simulink model "SiHADIR_Architecture"  (R2026a)
settings: Solver=VariableStepAuto
settings Model: DataDictionary=SiHADIR_Architecture_Interfaces.sldd  LastModifiedBy=Asus

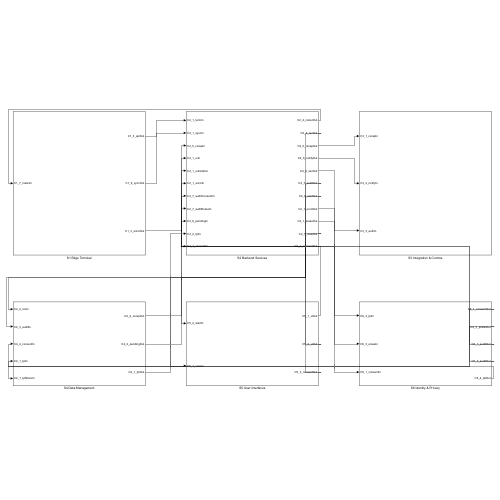
[thumbnail: Simulink's stored preview of the top-level diagram]
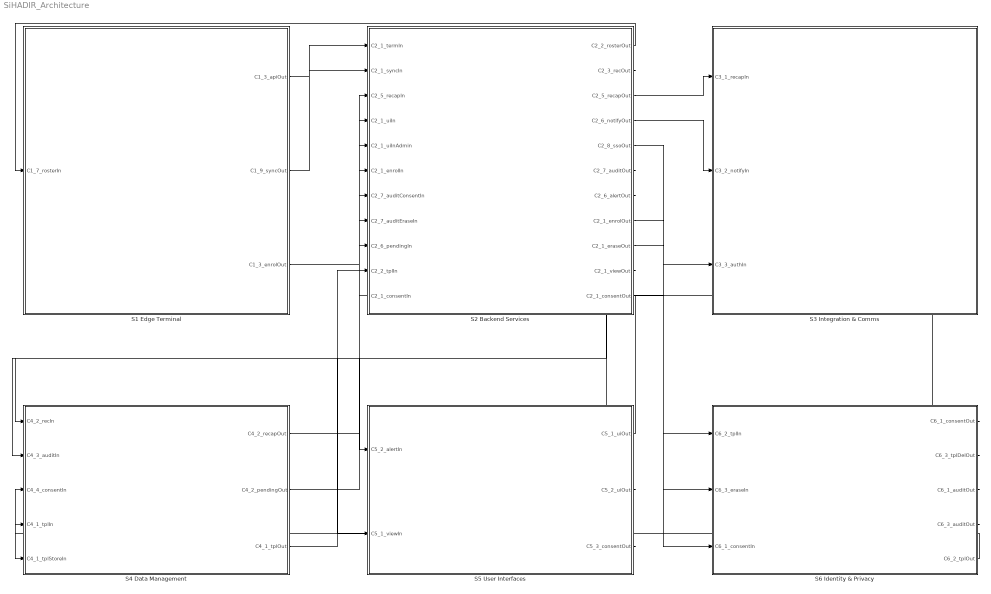
== system SiHADIR_Architecture ==
  S1 Edge Terminal : Subsystem  Description=Subsistem S1 | 11 komponen: C1.1, C1.2, C1.3, C1.4, C1.5, C1.6, C1.7, C1.8, C1.9, C1.10, C1.11
  S2 Backend Services : Subsystem  Description=Subsistem S2 | 8 komponen: C2.1, C2.2, C2.3, C2.4, C2.5, C2.6, C2.7, C2.8
  S3 Integration & Comms : Subsystem  Description=Subsistem S3 | 3 komponen: C3.1, C3.2, C3.3
  S4 Data Management : Subsystem  Description=Subsistem S4 | 4 komponen: C4.1, C4.2, C4.3, C4.4
  S5 User Interfaces : Subsystem  Description=Subsistem S5 | 3 komponen: C5.1, C5.2, C5.3
  S6 Identity & Privacy : Subsystem  Description=Subsistem S6 | 3 komponen: C6.1, C6.2, C6.3
  wires:
  S1 Edge Terminal/1(C1_3_apiOut) -> S2 Backend Services/1(C2_1_termIn)
  S1 Edge Terminal/2(C1_9_syncOut) -> S2 Backend Services/2(C2_1_syncIn)
  S2 Backend Services/1(C2_2_rosterOut) -> S1 Edge Terminal/1(C1_7_rosterIn)
  S2 Backend Services/2(C2_3_recOut) -> S4 Data Management/1(C4_2_recIn)
  S4 Data Management/1(C4_2_recapOut) -> S2 Backend Services/3(C2_5_recapIn)
  S2 Backend Services/3(C2_5_recapOut) -> S3 Integration & Comms/1(C3_1_recapIn)
  S2 Backend Services/4(C2_6_notifyOut) -> S3 Integration & Comms/2(C3_2_notifyIn)
  S2 Backend Services/5(C2_8_ssoOut) -> S3 Integration & Comms/3(C3_3_authIn)
  S2 Backend Services/6(C2_7_auditOut) -> S4 Data Management/2(C4_3_auditIn)
  S5 User Interfaces/1(C5_1_uiOut) -> S2 Backend Services/4(C2_1_uiIn)
  S5 User Interfaces/2(C5_2_uiOut) -> S2 Backend Services/5(C2_1_uiInAdmin)
  S6 Identity & Privacy/1(C6_1_consentOut) -> S4 Data Management/3(C4_4_consentIn)
  S6 Identity & Privacy/2(C6_3_tplDelOut) -> S4 Data Management/4(C4_1_tplIn)
  S1 Edge Terminal/3(C1_3_enrolOut) -> S2 Backend Services/6(C2_1_enrolIn)
  S6 Identity & Privacy/3(C6_1_auditOut) -> S2 Backend Services/7(C2_7_auditConsentIn)
  S6 Identity & Privacy/4(C6_3_auditOut) -> S2 Backend Services/8(C2_7_auditEraseIn)
  S4 Data Management/2(C4_2_pendingOut) -> S2 Backend Services/9(C2_6_pendingIn)
  S2 Backend Services/7(C2_6_alertOut) -> S5 User Interfaces/1(C5_2_alertIn)
  S2 Backend Services/8(C2_1_enrolOut) -> S6 Identity & Privacy/1(C6_2_tplIn)
  S6 Identity & Privacy/5(C6_2_tplOut) -> S4 Data Management/5(C4_1_tplStoreIn)
  S4 Data Management/3(C4_1_tplOut) -> S2 Backend Services/10(C2_2_tplIn)
  S2 Backend Services/9(C2_1_eraseOut) -> S6 Identity & Privacy/2(C6_3_eraseIn)
  S2 Backend Services/10(C2_1_viewOut) -> S5 User Interfaces/2(C5_1_viewIn)
  S5 User Interfaces/3(C5_3_consentOut) -> S2 Backend Services/11(C2_1_consentIn)
  S2 Backend Services/11(C2_1_consentOut) -> S6 Identity & Privacy/3(C6_1_consentIn)

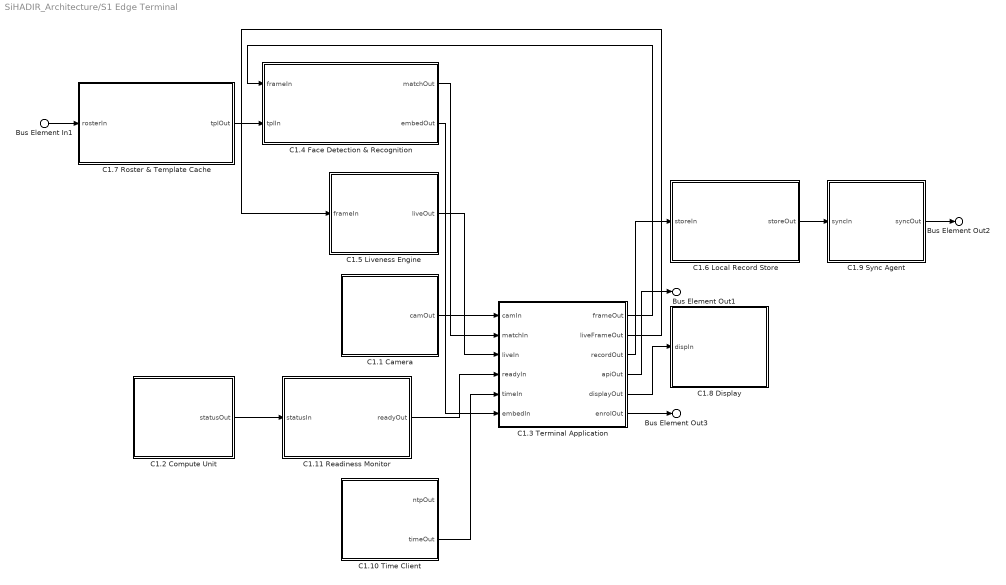
== system SiHADIR_Architecture/S1 Edge Terminal ==
  Bus Element In1 : Inport  PortName=C1_7_rosterIn
  C1.1 Camera : Subsystem  Description=ID=C1.1 | jenis=HW | fungsi=F2.1
  C1.10 Time Client : Subsystem  Description=ID=C1.10 | jenis=SW | fungsi=F12
  C1.11 Readiness Monitor : Subsystem  Description=ID=C1.11 | jenis=SW | fungsi=F11
  C1.2 Compute Unit : Subsystem  Description=ID=C1.2 | jenis=HW | fungsi=F2.2,F2.3,F2.4,F2.5,F11
  C1.3 Terminal Application : Subsystem  Description=ID=C1.3 | jenis=SW | fungsi=F3,F10
  C1.4 Face Detection & Recognition : Subsystem  Description=ID=C1.4 | jenis=SW/ML | fungsi=F2.2,F2.4,F2.5
  C1.5 Liveness Engine : Subsystem  Description=ID=C1.5 | jenis=SW/ML | fungsi=F2.3
  C1.6 Local Record Store : Subsystem  Description=ID=C1.6 | jenis=SW | fungsi=F4.2
  C1.7 Roster & Template Cache : Subsystem  Description=ID=C1.7 | jenis=SW | fungsi=F1.1,F2.5
  C1.8 Display : Subsystem  Description=ID=C1.8 | jenis=HW/SW | fungsi=F10
  C1.9 Sync Agent : Subsystem  Description=ID=C1.9 | jenis=SW | fungsi=F4.3
  Bus Element Out1 : Outport  PortName=C1_3_apiOut
  Bus Element Out2 : Outport  Port=2  PortName=C1_9_syncOut
  Bus Element Out3 : Outport  Port=3  PortName=C1_3_enrolOut
  wires:
  C1.6 Local Record Store/1(storeOut) -> C1.9 Sync Agent/1(syncIn)
  Bus Element In1/1 -> C1.7 Roster & Template Cache/1(rosterIn)
  C1.1 Camera/1(camOut) -> C1.3 Terminal Application/1(camIn)
  C1.5 Liveness Engine/1(liveOut) -> C1.3 Terminal Application/3(liveIn)
  C1.7 Roster & Template Cache/1(tplOut) -> C1.4 Face Detection & Recognition/2(tplIn)
  C1.2 Compute Unit/1(statusOut) -> C1.11 Readiness Monitor/1(statusIn)
  C1.11 Readiness Monitor/1(readyOut) -> C1.3 Terminal Application/4(readyIn)
  C1.4 Face Detection & Recognition/1(matchOut) -> C1.3 Terminal Application/2(matchIn)
  C1.4 Face Detection & Recognition/2(embedOut) -> C1.3 Terminal Application/6(embedIn)
  C1.10 Time Client/2(timeOut) -> C1.3 Terminal Application/5(timeIn)
  C1.3 Terminal Application/1(frameOut) -> C1.4 Face Detection & Recognition/1(frameIn)
  C1.3 Terminal Application/2(liveFrameOut) -> C1.5 Liveness Engine/1(frameIn)
  C1.3 Terminal Application/5(displayOut) -> C1.8 Display/1(dispIn)
  C1.3 Terminal Application/3(recordOut) -> C1.6 Local Record Store/1(storeIn)
  C1.3 Terminal Application/4(apiOut) -> Bus Element Out1/1
  C1.3 Terminal Application/6(enrolOut) -> Bus Element Out3/1
  C1.9 Sync Agent/1(syncOut) -> Bus Element Out2/1

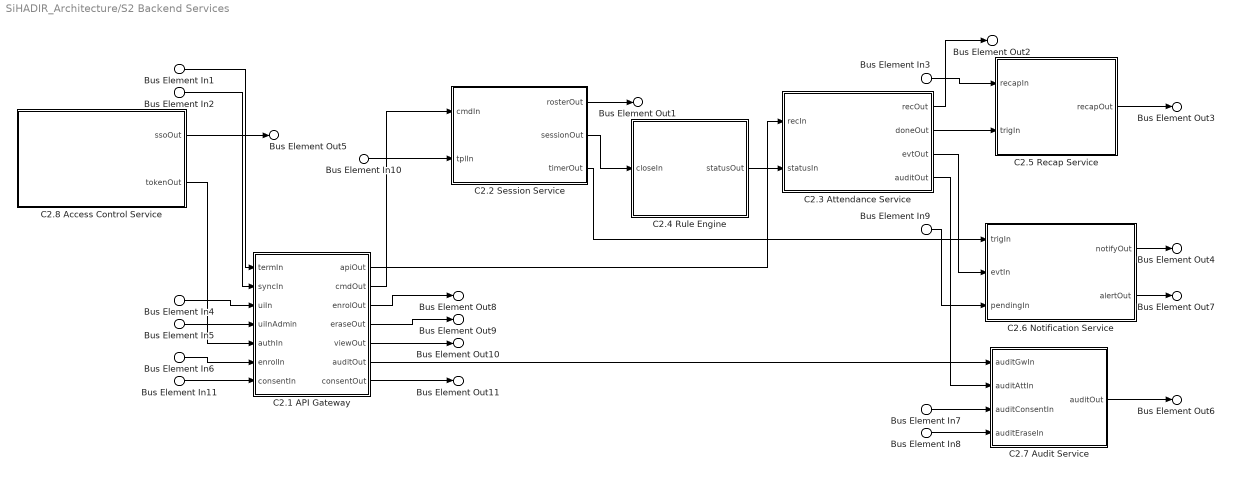
== system SiHADIR_Architecture/S2 Backend Services ==
  Bus Element In1 : Inport  PortName=C2_1_termIn
  Bus Element In2 : Inport  Port=2  PortName=C2_1_syncIn
  Bus Element In3 : Inport  Port=3  PortName=C2_5_recapIn
  Bus Element In4 : Inport  Port=4  PortName=C2_1_uiIn
  Bus Element In5 : Inport  Port=5  PortName=C2_1_uiInAdmin
  Bus Element In6 : Inport  Port=6  PortName=C2_1_enrolIn
  Bus Element In7 : Inport  Port=7  PortName=C2_7_auditConsentIn
  Bus Element In8 : Inport  Port=8  PortName=C2_7_auditEraseIn
  Bus Element In9 : Inport  Port=9  PortName=C2_6_pendingIn
  Bus Element In10 : Inport  Port=10  PortName=C2_2_tplIn
  Bus Element In11 : Inport  Port=11  PortName=C2_1_consentIn
  C2.1 API Gateway : Subsystem  Description=ID=C2.1 | jenis=SW | fungsi=F8.2
  C2.2 Session Service : Subsystem  Description=ID=C2.2 | jenis=SW | fungsi=F1.1,F1.2
  C2.3 Attendance Service : Subsystem  Description=ID=C2.3 | jenis=SW | fungsi=F4.1
  C2.4 Rule Engine : Subsystem  Description=ID=C2.4 | jenis=SW | fungsi=F3
  C2.5 Recap Service : Subsystem  Description=ID=C2.5 | jenis=SW | fungsi=F5.1,F5.2
  C2.6 Notification Service : Subsystem  Description=ID=C2.6 | jenis=SW | fungsi=F6.1,F6.2
  C2.7 Audit Service : Subsystem  Description=ID=C2.7 | jenis=SW | fungsi=F9
  C2.8 Access Control Service : Subsystem  Description=ID=C2.8 | jenis=SW | fungsi=F8.1
  Bus Element Out1 : Outport  PortName=C2_2_rosterOut
  Bus Element Out2 : Outport  Port=2  PortName=C2_3_recOut
  Bus Element Out3 : Outport  Port=3  PortName=C2_5_recapOut
  Bus Element Out4 : Outport  Port=4  PortName=C2_6_notifyOut
  Bus Element Out5 : Outport  Port=5  PortName=C2_8_ssoOut
  Bus Element Out6 : Outport  Port=6  PortName=C2_7_auditOut
  Bus Element Out7 : Outport  Port=7  PortName=C2_6_alertOut
  Bus Element Out8 : Outport  Port=8  PortName=C2_1_enrolOut
  Bus Element Out9 : Outport  Port=9  PortName=C2_1_eraseOut
  Bus Element Out10 : Outport  Port=10  PortName=C2_1_viewOut
  Bus Element Out11 : Outport  Port=11  PortName=C2_1_consentOut
  wires:
  Bus Element In2/1 -> C2.1 API Gateway/2(syncIn)
  Bus Element In4/1 -> C2.1 API Gateway/3(uiIn)
  Bus Element In6/1 -> C2.1 API Gateway/6(enrolIn)
  Bus Element In3/1 -> C2.5 Recap Service/1(recapIn)
  Bus Element In1/1 -> C2.1 API Gateway/1(termIn)
  Bus Element In5/1 -> C2.1 API Gateway/4(uiInAdmin)
  Bus Element In7/1 -> C2.7 Audit Service/3(auditConsentIn)
  Bus Element In9/1 -> C2.6 Notification Service/3(pendingIn)
  Bus Element In11/1 -> C2.1 API Gateway/7(consentIn)
  C2.8 Access Control Service/2(tokenOut) -> C2.1 API Gateway/5(authIn)
  C2.8 Access Control Service/1(ssoOut) -> Bus Element Out5/1
  Bus Element In10/1 -> C2.2 Session Service/2(tplIn)
  C2.1 API Gateway/5(viewOut) -> Bus Element Out10/1
  C2.1 API Gateway/1(apiOut) -> C2.3 Attendance Service/1(recIn)
  C2.1 API Gateway/6(auditOut) -> C2.7 Audit Service/1(auditGwIn)
  C2.1 API Gateway/2(cmdOut) -> C2.2 Session Service/1(cmdIn)
  C2.1 API Gateway/7(consentOut) -> Bus Element Out11/1
  C2.1 API Gateway/3(enrolOut) -> Bus Element Out8/1
  C2.1 API Gateway/4(eraseOut) -> Bus Element Out9/1
  C2.2 Session Service/1(rosterOut) -> Bus Element Out1/1
  C2.2 Session Service/2(sessionOut) -> C2.4 Rule Engine/1(closeIn)
  C2.2 Session Service/3(timerOut) -> C2.6 Notification Service/1(trigIn)
  C2.4 Rule Engine/1(statusOut) -> C2.3 Attendance Service/2(statusIn)
  C2.3 Attendance Service/1(recOut) -> Bus Element Out2/1
  C2.3 Attendance Service/2(doneOut) -> C2.5 Recap Service/2(trigIn)
  C2.3 Attendance Service/3(evtOut) -> C2.6 Notification Service/2(evtIn)
  C2.3 Attendance Service/4(auditOut) -> C2.7 Audit Service/2(auditAttIn)
  Bus Element In8/1 -> C2.7 Audit Service/4(auditEraseIn)
  C2.5 Recap Service/1(recapOut) -> Bus Element Out3/1
  C2.6 Notification Service/1(notifyOut) -> Bus Element Out4/1
  C2.6 Notification Service/2(alertOut) -> Bus Element Out7/1
  C2.7 Audit Service/1(auditOut) -> Bus Element Out6/1

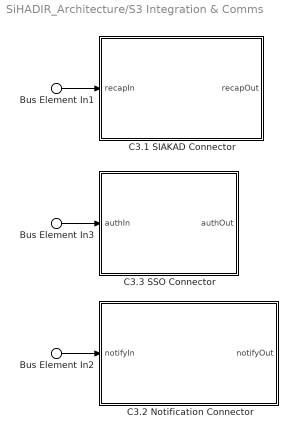
== system SiHADIR_Architecture/S3 Integration & Comms ==
  Bus Element In1 : Inport  PortName=C3_1_recapIn
  Bus Element In2 : Inport  Port=2  PortName=C3_2_notifyIn
  Bus Element In3 : Inport  Port=3  PortName=C3_3_authIn
  C3.1 SIAKAD Connector : Subsystem  Description=ID=C3.1 | jenis=SW | fungsi=F5.2
  C3.2 Notification Connector : Subsystem  Description=ID=C3.2 | jenis=SW | fungsi=F6.1
  C3.3 SSO Connector : Subsystem  Description=ID=C3.3 | jenis=SW | fungsi=F8.1
  wires:
  Bus Element In2/1 -> C3.2 Notification Connector/1(notifyIn)
  Bus Element In3/1 -> C3.3 SSO Connector/1(authIn)
  Bus Element In1/1 -> C3.1 SIAKAD Connector/1(recapIn)

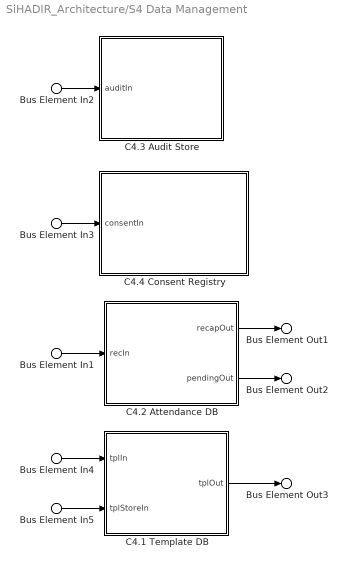
== system SiHADIR_Architecture/S4 Data Management ==
  Bus Element In1 : Inport  PortName=C4_2_recIn
  Bus Element In2 : Inport  Port=2  PortName=C4_3_auditIn
  Bus Element In3 : Inport  Port=3  PortName=C4_4_consentIn
  Bus Element In4 : Inport  Port=4  PortName=C4_1_tplIn
  Bus Element In5 : Inport  Port=5  PortName=C4_1_tplStoreIn
  C4.1 Template DB : Subsystem  Description=ID=C4.1 | jenis=Data | fungsi=F2.5,F7.2,F7.3
  C4.2 Attendance DB : Subsystem  Description=ID=C4.2 | jenis=Data | fungsi=F4.1,F5.1
  C4.3 Audit Store : Subsystem  Description=ID=C4.3 | jenis=Data | fungsi=F7.3,F9
  C4.4 Consent Registry : Subsystem  Description=ID=C4.4 | jenis=Data | fungsi=F7.1
  Bus Element Out1 : Outport  PortName=C4_2_recapOut
  Bus Element Out2 : Outport  Port=2  PortName=C4_2_pendingOut
  Bus Element Out3 : Outport  Port=3  PortName=C4_1_tplOut
  wires:
  C4.1 Template DB/1(tplOut) -> Bus Element Out3/1
  Bus Element In5/1 -> C4.1 Template DB/2(tplStoreIn)
  Bus Element In4/1 -> C4.1 Template DB/1(tplIn)
  Bus Element In1/1 -> C4.2 Attendance DB/1(recIn)
  Bus Element In3/1 -> C4.4 Consent Registry/1(consentIn)
  Bus Element In2/1 -> C4.3 Audit Store/1(auditIn)
  C4.2 Attendance DB/2(pendingOut) -> Bus Element Out2/1
  C4.2 Attendance DB/1(recapOut) -> Bus Element Out1/1

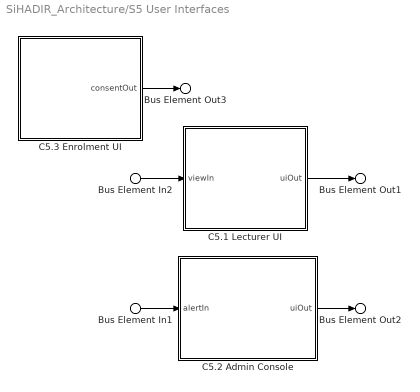
== system SiHADIR_Architecture/S5 User Interfaces ==
  Bus Element In1 : Inport  PortName=C5_2_alertIn
  Bus Element In2 : Inport  Port=2  PortName=C5_1_viewIn
  C5.1 Lecturer UI : Subsystem  Description=ID=C5.1 | jenis=SW | fungsi=F1.1,F1.2,F10
  C5.2 Admin Console : Subsystem  Description=ID=C5.2 | jenis=SW | fungsi=F6.2,F7.3
  C5.3 Enrolment UI : Subsystem  Description=ID=C5.3 | jenis=SW | fungsi=F7.1,F7.2
  Bus Element Out1 : Outport  PortName=C5_1_uiOut
  Bus Element Out2 : Outport  Port=2  PortName=C5_2_uiOut
  Bus Element Out3 : Outport  Port=3  PortName=C5_3_consentOut
  wires:
  C5.2 Admin Console/1(uiOut) -> Bus Element Out2/1
  C5.1 Lecturer UI/1(uiOut) -> Bus Element Out1/1
  Bus Element In1/1 -> C5.2 Admin Console/1(alertIn)
  Bus Element In2/1 -> C5.1 Lecturer UI/1(viewIn)
  C5.3 Enrolment UI/1(consentOut) -> Bus Element Out3/1

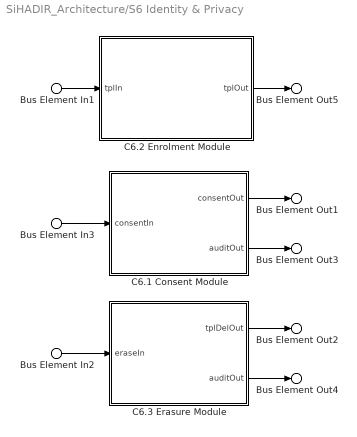
== system SiHADIR_Architecture/S6 Identity & Privacy ==
  Bus Element In1 : Inport  PortName=C6_2_tplIn
  Bus Element In2 : Inport  Port=2  PortName=C6_3_eraseIn
  Bus Element In3 : Inport  Port=3  PortName=C6_1_consentIn
  C6.1 Consent Module : Subsystem  Description=ID=C6.1 | jenis=SW | fungsi=F7.1
  C6.2 Enrolment Module : Subsystem  Description=ID=C6.2 | jenis=SW | fungsi=F7.2
  C6.3 Erasure Module : Subsystem  Description=ID=C6.3 | jenis=SW | fungsi=F7.3
  Bus Element Out1 : Outport  PortName=C6_1_consentOut
  Bus Element Out2 : Outport  Port=2  PortName=C6_3_tplDelOut
  Bus Element Out3 : Outport  Port=3  PortName=C6_1_auditOut
  Bus Element Out4 : Outport  Port=4  PortName=C6_3_auditOut
  Bus Element Out5 : Outport  Port=5  PortName=C6_2_tplOut
  wires:
  C6.1 Consent Module/2(auditOut) -> Bus Element Out3/1
  C6.1 Consent Module/1(consentOut) -> Bus Element Out1/1
  Bus Element In2/1 -> C6.3 Erasure Module/1(eraseIn)
  Bus Element In3/1 -> C6.1 Consent Module/1(consentIn)
  Bus Element In1/1 -> C6.2 Enrolment Module/1(tplIn)
  C6.3 Erasure Module/2(auditOut) -> Bus Element Out4/1
  C6.3 Erasure Module/1(tplDelOut) -> Bus Element Out2/1
  C6.2 Enrolment Module/1(tplOut) -> Bus Element Out5/1

== system SiHADIR_Architecture/S1 Edge Terminal/C1.1 Camera ==
  Bus Element Out1 : Outport  PortName=camOut

== system SiHADIR_Architecture/S1 Edge Terminal/C1.10 Time Client ==
  Bus Element Out1 : Outport  PortName=ntpOut
  Bus Element Out2 : Outport  Port=2  PortName=timeOut

== system SiHADIR_Architecture/S1 Edge Terminal/C1.11 Readiness Monitor ==
  Bus Element In1 : Inport  PortName=statusIn
  Bus Element Out1 : Outport  PortName=readyOut

== system SiHADIR_Architecture/S1 Edge Terminal/C1.2 Compute Unit ==
  Bus Element Out1 : Outport  PortName=statusOut

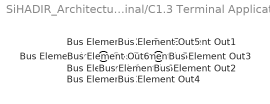
== system SiHADIR_Architecture/S1 Edge Terminal/C1.3 Terminal Application ==
  Bus Element In1 : Inport  PortName=camIn
  Bus Element In2 : Inport  Port=2  PortName=matchIn
  Bus Element In3 : Inport  Port=3  PortName=liveIn
  Bus Element In4 : Inport  Port=4  PortName=readyIn
  Bus Element In5 : Inport  Port=5  PortName=timeIn
  Bus Element In6 : Inport  Port=6  PortName=embedIn
  Bus Element Out1 : Outport  PortName=frameOut
  Bus Element Out2 : Outport  Port=2  PortName=liveFrameOut
  Bus Element Out3 : Outport  Port=3  PortName=recordOut
  Bus Element Out4 : Outport  Port=4  PortName=apiOut
  Bus Element Out5 : Outport  Port=5  PortName=displayOut
  Bus Element Out6 : Outport  Port=6  PortName=enrolOut

== system SiHADIR_Architecture/S1 Edge Terminal/C1.4 Face Detection & Recognition ==
  Bus Element In1 : Inport  PortName=frameIn
  Bus Element In2 : Inport  Port=2  PortName=tplIn
  Bus Element Out1 : Outport  PortName=matchOut
  Bus Element Out2 : Outport  Port=2  PortName=embedOut

== system SiHADIR_Architecture/S1 Edge Terminal/C1.5 Liveness Engine ==
  Bus Element In1 : Inport  PortName=frameIn
  Bus Element Out1 : Outport  PortName=liveOut

== system SiHADIR_Architecture/S1 Edge Terminal/C1.6 Local Record Store ==
  Bus Element In1 : Inport  PortName=storeIn
  Bus Element Out1 : Outport  PortName=storeOut

== system SiHADIR_Architecture/S1 Edge Terminal/C1.7 Roster & Template Cache ==
  Bus Element In1 : Inport  PortName=rosterIn
  Bus Element Out1 : Outport  PortName=tplOut

== system SiHADIR_Architecture/S1 Edge Terminal/C1.8 Display ==
  Bus Element In1 : Inport  PortName=dispIn

== system SiHADIR_Architecture/S1 Edge Terminal/C1.9 Sync Agent ==
  Bus Element In1 : Inport  PortName=syncIn
  Bus Element Out1 : Outport  PortName=syncOut

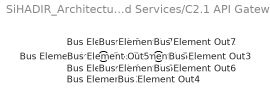
== system SiHADIR_Architecture/S2 Backend Services/C2.1 API Gateway ==
  Bus Element In1 : Inport  PortName=termIn
  Bus Element In2 : Inport  Port=2  PortName=syncIn
  Bus Element In3 : Inport  Port=3  PortName=uiIn
  Bus Element In4 : Inport  Port=4  PortName=uiInAdmin
  Bus Element In5 : Inport  Port=5  PortName=authIn
  Bus Element In6 : Inport  Port=6  PortName=enrolIn
  Bus Element In7 : Inport  Port=7  PortName=consentIn
  Bus Element Out1 : Outport  PortName=apiOut
  Bus Element Out2 : Outport  Port=2  PortName=cmdOut
  Bus Element Out3 : Outport  Port=3  PortName=enrolOut
  Bus Element Out4 : Outport  Port=4  PortName=eraseOut
  Bus Element Out5 : Outport  Port=5  PortName=viewOut
  Bus Element Out6 : Outport  Port=6  PortName=auditOut
  Bus Element Out7 : Outport  Port=7  PortName=consentOut

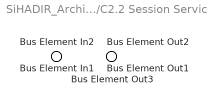
== system SiHADIR_Architecture/S2 Backend Services/C2.2 Session Service ==
  Bus Element In1 : Inport  PortName=cmdIn
  Bus Element In2 : Inport  Port=2  PortName=tplIn
  Bus Element Out1 : Outport  PortName=rosterOut
  Bus Element Out2 : Outport  Port=2  PortName=sessionOut
  Bus Element Out3 : Outport  Port=3  PortName=timerOut

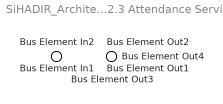
== system SiHADIR_Architecture/S2 Backend Services/C2.3 Attendance Service ==
  Bus Element In1 : Inport  PortName=recIn
  Bus Element In2 : Inport  Port=2  PortName=statusIn
  Bus Element Out1 : Outport  PortName=recOut
  Bus Element Out2 : Outport  Port=2  PortName=doneOut
  Bus Element Out3 : Outport  Port=3  PortName=evtOut
  Bus Element Out4 : Outport  Port=4  PortName=auditOut

== system SiHADIR_Architecture/S2 Backend Services/C2.4 Rule Engine ==
  Bus Element In1 : Inport  PortName=closeIn
  Bus Element Out1 : Outport  PortName=statusOut

== system SiHADIR_Architecture/S2 Backend Services/C2.5 Recap Service ==
  Bus Element In1 : Inport  PortName=recapIn
  Bus Element In2 : Inport  Port=2  PortName=trigIn
  Bus Element Out1 : Outport  PortName=recapOut

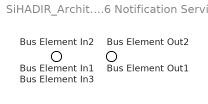
== system SiHADIR_Architecture/S2 Backend Services/C2.6 Notification Service ==
  Bus Element In1 : Inport  PortName=trigIn
  Bus Element In2 : Inport  Port=2  PortName=evtIn
  Bus Element In3 : Inport  Port=3  PortName=pendingIn
  Bus Element Out1 : Outport  PortName=notifyOut
  Bus Element Out2 : Outport  Port=2  PortName=alertOut

== system SiHADIR_Architecture/S2 Backend Services/C2.7 Audit Service ==
  Bus Element In1 : Inport  PortName=auditGwIn
  Bus Element In2 : Inport  Port=2  PortName=auditAttIn
  Bus Element In3 : Inport  Port=3  PortName=auditConsentIn
  Bus Element In4 : Inport  Port=4  PortName=auditEraseIn
  Bus Element Out1 : Outport  PortName=auditOut

== system SiHADIR_Architecture/S2 Backend Services/C2.8 Access Control Service ==
  Bus Element Out1 : Outport  PortName=ssoOut
  Bus Element Out2 : Outport  Port=2  PortName=tokenOut

== system SiHADIR_Architecture/S3 Integration & Comms/C3.1 SIAKAD Connector ==
  Bus Element In1 : Inport  PortName=recapIn
  Bus Element Out1 : Outport  PortName=recapOut

== system SiHADIR_Architecture/S3 Integration & Comms/C3.2 Notification Connector ==
  Bus Element In1 : Inport  PortName=notifyIn
  Bus Element Out1 : Outport  PortName=notifyOut

== system SiHADIR_Architecture/S3 Integration & Comms/C3.3 SSO Connector ==
  Bus Element In1 : Inport  PortName=authIn
  Bus Element Out1 : Outport  PortName=authOut

== system SiHADIR_Architecture/S4 Data Management/C4.1 Template DB ==
  Bus Element In1 : Inport  PortName=tplIn
  Bus Element In2 : Inport  Port=2  PortName=tplStoreIn
  Bus Element Out1 : Outport  PortName=tplOut

== system SiHADIR_Architecture/S4 Data Management/C4.2 Attendance DB ==
  Bus Element In1 : Inport  PortName=recIn
  Bus Element Out1 : Outport  PortName=recapOut
  Bus Element Out2 : Outport  Port=2  PortName=pendingOut

== system SiHADIR_Architecture/S4 Data Management/C4.3 Audit Store ==
  Bus Element In1 : Inport  PortName=auditIn

== system SiHADIR_Architecture/S4 Data Management/C4.4 Consent Registry ==
  Bus Element In1 : Inport  PortName=consentIn

== system SiHADIR_Architecture/S5 User Interfaces/C5.1 Lecturer UI ==
  Bus Element In1 : Inport  PortName=viewIn
  Bus Element Out1 : Outport  PortName=uiOut

== system SiHADIR_Architecture/S5 User Interfaces/C5.2 Admin Console ==
  Bus Element In1 : Inport  PortName=alertIn
  Bus Element Out1 : Outport  PortName=uiOut

== system SiHADIR_Architecture/S5 User Interfaces/C5.3 Enrolment UI ==
  Bus Element Out1 : Outport  PortName=consentOut

== system SiHADIR_Architecture/S6 Identity & Privacy/C6.1 Consent Module ==
  Bus Element In1 : Inport  PortName=consentIn
  Bus Element Out1 : Outport  PortName=consentOut
  Bus Element Out2 : Outport  Port=2  PortName=auditOut

== system SiHADIR_Architecture/S6 Identity & Privacy/C6.2 Enrolment Module ==
  Bus Element In1 : Inport  PortName=tplIn
  Bus Element Out1 : Outport  PortName=tplOut

== system SiHADIR_Architecture/S6 Identity & Privacy/C6.3 Erasure Module ==
  Bus Element In1 : Inport  PortName=eraseIn
  Bus Element Out1 : Outport  PortName=tplDelOut
  Bus Element Out2 : Outport  Port=2  PortName=auditOut
